simulink model "Half_3_Legs_with_RL_load"  (R2025b)
settings: Solver=VariableStepAuto  StartTime=0.0  StopTime=0.1  FixedStep=1e-6  MaxStep=1e-6  RelTol=1e-4
values from neighbouring files (symbols this model uses):
  bias_current = 5    [parameters_for_AMB_topology.m]
  half_SW_Ts = SW_Ts*0.5    (= 2.5e-05)    [parameters_for_AMB_topology.m]
  K_i = 2*pi*f_c*R_value/U_dc    (= 47.1238898038)    [parameters_for_AMB_topology.m]
  K_p = 2*pi*f_c*L_value/U_dc    (= 0.0235619449019)    [parameters_for_AMB_topology.m]
  R_value = 1    [parameters_for_AMB_topology.m]
  SW_Ts = 1/(SW_frequency)    (= 5e-05)    [parameters_for_AMB_topology.m]
libraries: fl_lib x48, simulink x35, nesl_utility x26, ee_lib x16, eeGeneralControl x10
(part 1 of 4)
settings Model: SimulationMode=accelerator  Creator=ubuntu  LastModifiedBy=ubuntu

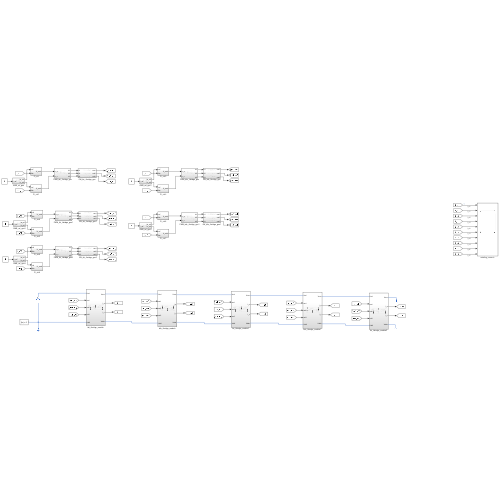
[thumbnail: Simulink's stored preview of the top-level diagram]
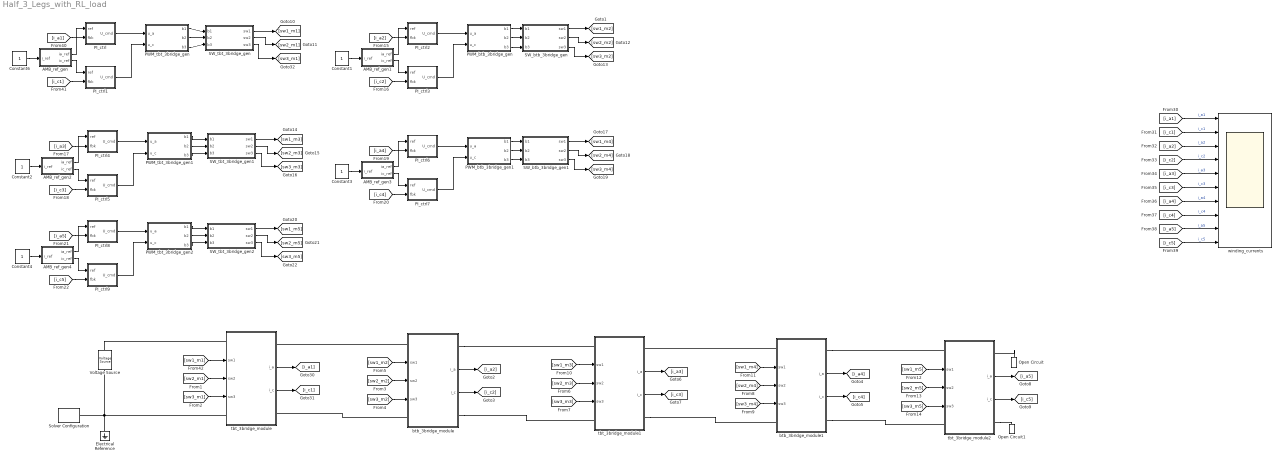
== system Half_3_Legs_with_RL_load ==
  AMB_ref_gen : Subsystem
  AMB_ref_gen1 : Subsystem
  AMB_ref_gen2 : Subsystem
  AMB_ref_gen3 : Subsystem
  AMB_ref_gen4 : Subsystem
  Constant{1..4,6} (5 alike) : Constant
  Electrical Reference : fl_lib/Electrical/Electrical Elements/Electrical Reference
  Open Circuit : fl_lib/Electrical/Electrical Elements/Open Circuit  v_specify=off  v_priority=None  v=0 V  v_nominal_specify=off  v_nominal_value=1  v_nominal_unit=V
  Open Circuit1 : fl_lib/Electrical/Electrical Elements/Open Circuit  v_specify=off  v_priority=None  v=0 V  v_nominal_specify=off  v_nominal_value=1  v_nominal_unit=V
  PI_ctrl : Subsystem
  PI_ctrl1 : Subsystem
  PI_ctrl2 : Subsystem
  PI_ctrl3 : Subsystem
  PI_ctrl4 : Subsystem
  PI_ctrl5 : Subsystem
  PI_ctrl6 : Subsystem
  PI_ctrl7 : Subsystem
  PI_ctrl8 : Subsystem
  PI_ctrl9 : Subsystem
  PWM_btb_3bridge_gen : Subsystem
  PWM_btb_3bridge_gen1 : Subsystem
  PWM_tbt_3bridge_gen : Subsystem
  PWM_tbt_3bridge_gen1 : Subsystem
  PWM_tbt_3bridge_gen2 : Subsystem
  SW_btb_3bridge_gen : Subsystem
  SW_btb_3bridge_gen1 : Subsystem
  SW_tbt_3bridge_gen : Subsystem
  SW_tbt_3bridge_gen1 : Subsystem
  SW_tbt_3bridge_gen2 : Subsystem
  Solver Configuration : nesl_utility/Solver Configuration  PhysicalDomain=network_engine_domain  SubClassName=solver  LeftPortType=input  RightPortType=generic  Tones=[]  Harmonics=[]  SimulateNoise=off  Profile=off  UseLocalSampling=off  EnableSwitchedLinearOptims=on  FrequencyDomain=off  UseCCode=off  RelTol=0.001  AbsTol=0.001  MinStep=1e-09  ToWorkspace=off  RevertToSquareIcSolve=off  NumHomotopyIterations=100  PhasorMode=off  PhasorModeNumHarmonics=1  ConsistencySolver=NEWTON_XTOL_AFTER_FTOL  IndexReductionMethod=DerivativeReplacement  DoDC=off  ResidualTolerance=1e-09  ConsistencyTolSource=GLOBAL  ConsistencyAbsTol=0.001  ConsistencyRelTol=0.001  ConsistencyTolFactor=0.001  UseLocalSolver=off  LocalSolverChoice=NE_TRAPEZOIDAL_ADVANCER  ResolveIndetEquations=on  FunctionEvalNumThread=1  LocalSolverSampleTime=1e-6  DoFixedCost=off  MaxNonlinIter=3  MaxModeIter=2  ComputeImpulses=off  ImpulseIterations=2  LinearAlgebra=auto  LinearAlgebraNumThread=0  EquationFormulation=NE_TIME_EF  DelaysMemoryBudget=1024  AutomaticFiltering=on  FilteringTimeConstant=0.001  PartitionStorageMethod=AS_NEEDED  PartitionMemoryBudget=1024  PartitionMethod=ROBUST  MultibodyUseLocalSolver=off  MultibodyLocalSolverChoice=ODE1  MultibodyLocalSolverSampleTime=0.001
  Voltage Source : ee_lib/Sources/Voltage Source  dc_voltage=U_dc V  ac_voltage=0 V  ac_shift=0 rad  ac_frequency=60 Hz  noise_mode=ee.enum.sources.noise.Disabled  PSD=0 V^2/Hz  sample_time=1e-3 s  repeatability=ee.enum.sources.repeatability.NotRepeatable  user_seed=0  auto_seed=3499211588  i_specify=off  i_priority=None  i=0 A  i_nominal_specify=off  i_nominal_value=1  i_nominal_unit=A  v_specify=off  v_priority=None  v=0 V  v_nominal_specify=off  v_nominal_value=1  v_nominal_unit=V
  btb_3bridge_module : Subsystem
      settings: PortSchema="{\"entries\":[{\"content\":{\"sides\":[{\"content\":{\"connectorIds\":[\"LConn1\",\"In1\",\"In2\",\"In3\",\"LConn2\"]},\"type\":\"ConnectorPlacement.EquallySpacedRectSide\",\"uuid\":\"10840d64-2819-4406-b8bd-231f9b995eba\"},{\"content\":{\"connectorIds\":[\"RConn1\",\"Out1\",\"Out2\",\"RConn2\"],\"side\":\"RIGHT\"},\"type\":\"ConnectorPlacement.EquallySpacedRectSide\",\"uuid\":\"cbdb59db-7701-4ec8-b1d6-0cae4f1e7bab\"},{\"content\":{\"side\":\"TOP\"},\"type\":\"ConnectorPlacement.EquallySpacedRectSide\",\"uuid\":\"7d2d29df-036d-4b8e-bd54-59e76fc95f5a\"}]},\"type\":\"ConnectorPlacement.EquallySpacedConnector\",\"uuid\":\"03b861fb-a6f3-4cde-b4d6-1419ababfbe2\"}],\"packageUris\":[\"http://schema.mathworks.com/mf0/Connector/R2020b\"],\"version\":\"1.0\"}"
  btb_3bridge_module1 : Subsystem
      settings: PortSchema="{\"entries\":[{\"content\":{\"sides\":[{\"content\":{\"connectorIds\":[\"LConn1\",\"In1\",\"In2\",\"In3\",\"LConn2\"]},\"type\":\"ConnectorPlacement.EquallySpacedRectSide\",\"uuid\":\"10840d64-2819-4406-b8bd-231f9b995eba\"},{\"content\":{\"connectorIds\":[\"RConn1\",\"Out1\",\"Out2\",\"RConn2\"],\"side\":\"RIGHT\"},\"type\":\"ConnectorPlacement.EquallySpacedRectSide\",\"uuid\":\"cbdb59db-7701-4ec8-b1d6-0cae4f1e7bab\"},{\"content\":{\"side\":\"TOP\"},\"type\":\"ConnectorPlacement.EquallySpacedRectSide\",\"uuid\":\"7d2d29df-036d-4b8e-bd54-59e76fc95f5a\"}]},\"type\":\"ConnectorPlacement.EquallySpacedConnector\",\"uuid\":\"03b861fb-a6f3-4cde-b4d6-1419ababfbe2\"}],\"packageUris\":[\"http://schema.mathworks.com/mf0/Connector/R2020b\"],\"version\":\"1.0\"}"
  tbt_3bridge_module : Subsystem
      settings: PortSchema="{\"entries\":[{\"content\":{\"sides\":[{\"content\":{\"connectorIds\":[\"LConn1\",\"In1\",\"In2\",\"In3\",\"LConn2\"]},\"type\":\"ConnectorPlacement.EquallySpacedRectSide\",\"uuid\":\"10840d64-2819-4406-b8bd-231f9b995eba\"},{\"content\":{\"connectorIds\":[\"RConn1\",\"Out1\",\"Out2\",\"RConn2\"],\"side\":\"RIGHT\"},\"type\":\"ConnectorPlacement.EquallySpacedRectSide\",\"uuid\":\"cbdb59db-7701-4ec8-b1d6-0cae4f1e7bab\"},{\"content\":{\"side\":\"TOP\"},\"type\":\"ConnectorPlacement.EquallySpacedRectSide\",\"uuid\":\"7d2d29df-036d-4b8e-bd54-59e76fc95f5a\"}]},\"type\":\"ConnectorPlacement.EquallySpacedConnector\",\"uuid\":\"03b861fb-a6f3-4cde-b4d6-1419ababfbe2\"}],\"packageUris\":[\"http://schema.mathworks.com/mf0/Connector/R2020b\"],\"version\":\"1.0\"}"
  tbt_3bridge_module1 : Subsystem
      settings: PortSchema="{\"entries\":[{\"content\":{\"sides\":[{\"content\":{\"connectorIds\":[\"LConn1\",\"In1\",\"In2\",\"In3\",\"LConn2\"]},\"type\":\"ConnectorPlacement.EquallySpacedRectSide\",\"uuid\":\"10840d64-2819-4406-b8bd-231f9b995eba\"},{\"content\":{\"connectorIds\":[\"RConn1\",\"Out1\",\"Out2\",\"RConn2\"],\"side\":\"RIGHT\"},\"type\":\"ConnectorPlacement.EquallySpacedRectSide\",\"uuid\":\"cbdb59db-7701-4ec8-b1d6-0cae4f1e7bab\"},{\"content\":{\"side\":\"TOP\"},\"type\":\"ConnectorPlacement.EquallySpacedRectSide\",\"uuid\":\"7d2d29df-036d-4b8e-bd54-59e76fc95f5a\"}]},\"type\":\"ConnectorPlacement.EquallySpacedConnector\",\"uuid\":\"03b861fb-a6f3-4cde-b4d6-1419ababfbe2\"}],\"packageUris\":[\"http://schema.mathworks.com/mf0/Connector/R2020b\"],\"version\":\"1.0\"}"
  tbt_3bridge_module2 : Subsystem
      settings: PortSchema="{\"entries\":[{\"content\":{\"sides\":[{\"content\":{\"connectorIds\":[\"LConn1\",\"In1\",\"In2\",\"In3\",\"LConn2\"]},\"type\":\"ConnectorPlacement.EquallySpacedRectSide\",\"uuid\":\"10840d64-2819-4406-b8bd-231f9b995eba\"},{\"content\":{\"connectorIds\":[\"RConn1\",\"Out1\",\"Out2\",\"RConn2\"],\"side\":\"RIGHT\"},\"type\":\"ConnectorPlacement.EquallySpacedRectSide\",\"uuid\":\"cbdb59db-7701-4ec8-b1d6-0cae4f1e7bab\"},{\"content\":{\"side\":\"TOP\"},\"type\":\"ConnectorPlacement.EquallySpacedRectSide\",\"uuid\":\"7d2d29df-036d-4b8e-bd54-59e76fc95f5a\"}]},\"type\":\"ConnectorPlacement.EquallySpacedConnector\",\"uuid\":\"03b861fb-a6f3-4cde-b4d6-1419ababfbe2\"}],\"packageUris\":[\"http://schema.mathworks.com/mf0/Connector/R2020b\"],\"version\":\"1.0\"}"
  winding_currents : Scope  NumInputPorts=10
      settings: ActiveDisplayYMinimum=-0.73222271304047026  ActiveDisplayYMaximum=6.5900064127702036
  wires:
  [i_a1] -> winding_currents/1  "i_a1"
  [i_c1] -> winding_currents/2  "i_c1"
  [i_a2] -> winding_currents/3  "i_a2"
  [i_c2] -> winding_currents/4  "i_c2"
  [i_a3] -> winding_currents/5  "i_a3"
  [i_c3] -> winding_currents/6  "i_c3"
  [i_a4] -> winding_currents/7  "i_a4"
  [i_c4] -> winding_currents/8  "i_c4"
  [i_a5] -> winding_currents/9  "i_a5"
  [i_c5] -> winding_currents/10  "i_c5"
  AMB_ref_gen/1(ia_ref) -> PI_ctrl/1(ref)
  AMB_ref_gen/2(ic_ref) -> PI_ctrl1/1(ref)
  Constant6/1 -> AMB_ref_gen/1(i_ref)
  [i_a1] -> PI_ctrl/2(fbk)
  [i_c1] -> PI_ctrl1/2(fbk)
  PI_ctrl/1(U_cmd) -> PWM_tbt_3bridge_gen/1(u_a)
  PI_ctrl1/1(U_cmd) -> PWM_tbt_3bridge_gen/2(u_c)
  PWM_tbt_3bridge_gen/1(b1) -> SW_tbt_3bridge_gen/1(b1)
  PWM_tbt_3bridge_gen/2(b2) -> SW_tbt_3bridge_gen/2(b2)
  PWM_tbt_3bridge_gen/3(b3) -> SW_tbt_3bridge_gen/3(b3)
  tbt_3bridge_module/1(i_a) -> [i_a1]
  tbt_3bridge_module/2(i_c) -> [i_c1]
  [sw1_m1] -> tbt_3bridge_module/1(sw1)
  [sw2_m1] -> tbt_3bridge_module/2(sw2)
  [sw3_m1] -> tbt_3bridge_module/3(sw3)
  [sw1_m2] -> btb_3bridge_module/1(sw1)
  [sw3_m2] -> btb_3bridge_module/3(sw3)
  [sw2_m2] -> btb_3bridge_module/2(sw2)
  btb_3bridge_module/1(i_a) -> [i_a2]
  btb_3bridge_module/2(i_c) -> [i_c2]
  [sw2_m4] -> btb_3bridge_module1/2(sw2)
  btb_3bridge_module1/1(i_a) -> [i_a4]
  [sw2_m3] -> tbt_3bridge_module1/2(sw2)
  [sw1_m4] -> btb_3bridge_module1/1(sw1)
  [sw1_m3] -> tbt_3bridge_module1/1(sw1)
  [sw3_m3] -> tbt_3bridge_module1/3(sw3)
  btb_3bridge_module1/2(i_c) -> [i_c4]
  [sw3_m4] -> btb_3bridge_module1/3(sw3)
  tbt_3bridge_module1/2(i_c) -> [i_c3]
  tbt_3bridge_module1/1(i_a) -> [i_a3]
  tbt_3bridge_module2/2(i_c) -> [i_c5]
  [sw3_m5] -> tbt_3bridge_module2/3(sw3)
  [sw2_m5] -> tbt_3bridge_module2/2(sw2)
  [sw1_m5] -> tbt_3bridge_module2/1(sw1)
  tbt_3bridge_module2/1(i_a) -> [i_a5]
  SW_tbt_3bridge_gen/1(sw1) -> [sw1_m1]
  SW_tbt_3bridge_gen/2(sw2) -> [sw2_m1]
  SW_tbt_3bridge_gen/3(sw3) -> [sw3_m1]
  [i_c2] -> PI_ctrl3/2(fbk)
  SW_btb_3bridge_gen/2(sw2) -> [sw2_m2]
  PWM_btb_3bridge_gen/2(b2) -> SW_btb_3bridge_gen/2(b2)
  PI_ctrl2/1(U_cmd) -> PWM_btb_3bridge_gen/1(u_a)
  AMB_ref_gen1/2(ic_ref) -> PI_ctrl3/1(ref)
  PWM_btb_3bridge_gen/1(b1) -> SW_btb_3bridge_gen/1(b1)
  AMB_ref_gen1/1(ia_ref) -> PI_ctrl2/1(ref)
  SW_btb_3bridge_gen/1(sw1) -> [sw1_m2]
  SW_btb_3bridge_gen/3(sw3) -> [sw3_m2]
  PI_ctrl3/1(U_cmd) -> PWM_btb_3bridge_gen/2(u_c)
  PWM_btb_3bridge_gen/3(b3) -> SW_btb_3bridge_gen/3(b3)
  [i_a2] -> PI_ctrl2/2(fbk)
  Constant1/1 -> AMB_ref_gen1/1(i_ref)
  [i_c3] -> PI_ctrl5/2(fbk)
  SW_tbt_3bridge_gen1/2(sw2) -> [sw2_m3]
  PWM_tbt_3bridge_gen1/2(b2) -> SW_tbt_3bridge_gen1/2(b2)
  PI_ctrl4/1(U_cmd) -> PWM_tbt_3bridge_gen1/1(u_a)
  AMB_ref_gen2/2(ic_ref) -> PI_ctrl5/1(ref)
  PWM_tbt_3bridge_gen1/1(b1) -> SW_tbt_3bridge_gen1/1(b1)
  AMB_ref_gen2/1(ia_ref) -> PI_ctrl4/1(ref)
  SW_tbt_3bridge_gen1/1(sw1) -> [sw1_m3]
  SW_tbt_3bridge_gen1/3(sw3) -> [sw3_m3]
  PI_ctrl5/1(U_cmd) -> PWM_tbt_3bridge_gen1/2(u_c)
  PWM_tbt_3bridge_gen1/3(b3) -> SW_tbt_3bridge_gen1/3(b3)
  [i_a3] -> PI_ctrl4/2(fbk)
  Constant2/1 -> AMB_ref_gen2/1(i_ref)
  AMB_ref_gen3/2(ic_ref) -> PI_ctrl7/1(ref)
  PWM_btb_3bridge_gen1/3(b3) -> SW_btb_3bridge_gen1/3(b3)
  SW_btb_3bridge_gen1/1(sw1) -> [sw1_m4]
  PWM_btb_3bridge_gen1/1(b1) -> SW_btb_3bridge_gen1/1(b1)
  SW_btb_3bridge_gen1/2(sw2) -> [sw2_m4]
  [i_c4] -> PI_ctrl7/2(fbk)
  AMB_ref_gen3/1(ia_ref) -> PI_ctrl6/1(ref)
  [i_a4] -> PI_ctrl6/2(fbk)
  SW_btb_3bridge_gen1/3(sw3) -> [sw3_m4]
  PWM_btb_3bridge_gen1/2(b2) -> SW_btb_3bridge_gen1/2(b2)
  PI_ctrl6/1(U_cmd) -> PWM_btb_3bridge_gen1/1(u_a)
  Constant3/1 -> AMB_ref_gen3/1(i_ref)
  PI_ctrl7/1(U_cmd) -> PWM_btb_3bridge_gen1/2(u_c)
  PWM_tbt_3bridge_gen2/2(b2) -> SW_tbt_3bridge_gen2/2(b2)
  PI_ctrl8/1(U_cmd) -> PWM_tbt_3bridge_gen2/1(u_a)
  SW_tbt_3bridge_gen2/1(sw1) -> [sw1_m5]
  [i_c5] -> PI_ctrl9/2(fbk)
  AMB_ref_gen4/2(ic_ref) -> PI_ctrl9/1(ref)
  PWM_tbt_3bridge_gen2/1(b1) -> SW_tbt_3bridge_gen2/1(b1)
  PWM_tbt_3bridge_gen2/3(b3) -> SW_tbt_3bridge_gen2/3(b3)
  AMB_ref_gen4/1(ia_ref) -> PI_ctrl8/1(ref)
  Constant4/1 -> AMB_ref_gen4/1(i_ref)
  PI_ctrl9/1(U_cmd) -> PWM_tbt_3bridge_gen2/2(u_c)
  SW_tbt_3bridge_gen2/3(sw3) -> [sw3_m5]
  [i_a5] -> PI_ctrl8/2(fbk)
  SW_tbt_3bridge_gen2/2(sw2) -> [sw2_m5]
  connections:
  Electrical Reference/LConn1 -- Voltage Source/RConn1 -- tbt_3bridge_module/LConn2 -- Solver Configuration/RConn1
  tbt_3bridge_module/LConn1 -- Voltage Source/LConn1
  btb_3bridge_module/LConn1 -- tbt_3bridge_module/RConn1
  btb_3bridge_module/LConn2 -- tbt_3bridge_module/RConn2
  btb_3bridge_module/RConn1 -- tbt_3bridge_module1/LConn1
  btb_3bridge_module/RConn2 -- tbt_3bridge_module1/LConn2
  btb_3bridge_module1/LConn1 -- tbt_3bridge_module1/RConn1
  tbt_3bridge_module1/RConn2 -- btb_3bridge_module1/LConn2
  btb_3bridge_module1/RConn1 -- tbt_3bridge_module2/LConn1
  btb_3bridge_module1/RConn2 -- tbt_3bridge_module2/LConn2
  Open Circuit/LConn1 -- tbt_3bridge_module2/RConn1
  tbt_3bridge_module2/RConn2 -- Open Circuit1/LConn1

== system Half_3_Legs_with_RL_load/AMB_ref_gen ==
  i_ref : Inport
  Add : Sum
  Add1 : Sum  Inputs=-+
  Constant : Constant  Value=bias_current
  Gain : Gain  Gain=0.5
  ia_ref : Outport
  ic_ref : Outport  Port=2
  wires:
  i_ref/1 -> Gain/1
  Gain/1 -> Add1/1, Add/2
  Add/1 -> ia_ref/1
  Constant/1 -> Add1/2, Add/1
  Add1/1 -> ic_ref/1

== system Half_3_Legs_with_RL_load/AMB_ref_gen1 ==
  i_ref : Inport
  Add : Sum
  Add1 : Sum  Inputs=-+
  Constant : Constant  Value=bias_current
  Gain : Gain  Gain=0.5
  ia_ref : Outport
  ic_ref : Outport  Port=2
  wires:
  i_ref/1 -> Gain/1
  Gain/1 -> Add1/1, Add/2
  Add/1 -> ia_ref/1
  Constant/1 -> Add1/2, Add/1
  Add1/1 -> ic_ref/1

== system Half_3_Legs_with_RL_load/AMB_ref_gen2 ==
  i_ref : Inport
  Add : Sum
  Add1 : Sum  Inputs=-+
  Constant : Constant  Value=bias_current
  Gain : Gain  Gain=0.5
  ia_ref : Outport
  ic_ref : Outport  Port=2
  wires:
  i_ref/1 -> Gain/1
  Gain/1 -> Add1/1, Add/2
  Add/1 -> ia_ref/1
  Constant/1 -> Add1/2, Add/1
  Add1/1 -> ic_ref/1

== system Half_3_Legs_with_RL_load/AMB_ref_gen3 ==
  i_ref : Inport
  Add : Sum
  Add1 : Sum  Inputs=-+
  Constant : Constant  Value=bias_current
  Gain : Gain  Gain=0.5
  ia_ref : Outport
  ic_ref : Outport  Port=2
  wires:
  i_ref/1 -> Gain/1
  Gain/1 -> Add1/1, Add/2
  Add/1 -> ia_ref/1
  Constant/1 -> Add1/2, Add/1
  Add1/1 -> ic_ref/1

== system Half_3_Legs_with_RL_load/AMB_ref_gen4 ==
  i_ref : Inport
  Add : Sum
  Add1 : Sum  Inputs=-+
  Constant : Constant  Value=bias_current
  Gain : Gain  Gain=0.5
  ia_ref : Outport
  ic_ref : Outport  Port=2
  wires:
  i_ref/1 -> Gain/1
  Gain/1 -> Add1/1, Add/2
  Add/1 -> ia_ref/1
  Constant/1 -> Add1/2, Add/1
  Add1/1 -> ic_ref/1

== system Half_3_Legs_with_RL_load/PI_ctrl ==
  ref : Inport
  fbk : Inport  Port=2
  Add2 : Sum  Inputs=+-
  Add3 : Sum
  Gain4 : Gain  Gain=K_p
  Ictrl_anti_windup : Subsystem
  Memory : Memory
  Rate Transition : RateTransition  OutPortSampleTime=SW_Ts
  Saturation : Saturate  UpperLimit=1  LowerLimit=-1
  Second-Order Filter : eeGeneralControl/Second-Order Filter  FilterType=Low-pass  fn=6000  Zeta=0.707  Ts=0  A0=0  Ph0=0  f0=0  b0=0
      settings: LibrarySourceBlock=ee_sl_lib/General Control/Second-Order Filter
  U_cmd : Outport
  wires:
  Gain4/1 -> Add3/1
  Memory/1 -> Second-Order Filter/1
  Second-Order Filter/1 -> Add2/2
  Saturation/1 -> U_cmd/1
  Add2/1 -> Ictrl_anti_windup/1(err), Gain4/1
  Add3/1 -> Saturation/1
  ref/1 -> Add2/1
  fbk/1 -> Rate Transition/1
  Rate Transition/1 -> Memory/1
  Ictrl_anti_windup/1(Int_out) -> Add3/2

== system Half_3_Legs_with_RL_load/PI_ctrl1 ==
  ref : Inport
  fbk : Inport  Port=2
  Add2 : Sum  Inputs=+-
  Add3 : Sum
  Gain4 : Gain  Gain=K_p
  Ictrl_anti_windup : Subsystem
  Memory : Memory
  Rate Transition : RateTransition  OutPortSampleTime=SW_Ts
  Saturation : Saturate  UpperLimit=1  LowerLimit=-1
  Second-Order Filter : eeGeneralControl/Second-Order Filter  FilterType=Low-pass  fn=6000  Zeta=0.707  Ts=0  A0=0  Ph0=0  f0=0  b0=0
      settings: LibrarySourceBlock=ee_sl_lib/General Control/Second-Order Filter
  U_cmd : Outport
  wires:
  Gain4/1 -> Add3/1
  Memory/1 -> Second-Order Filter/1
  Second-Order Filter/1 -> Add2/2
  Saturation/1 -> U_cmd/1
  Add2/1 -> Ictrl_anti_windup/1(err), Gain4/1
  Add3/1 -> Saturation/1
  ref/1 -> Add2/1
  fbk/1 -> Rate Transition/1
  Rate Transition/1 -> Memory/1
  Ictrl_anti_windup/1(Int_out) -> Add3/2

== system Half_3_Legs_with_RL_load/PI_ctrl2 ==
  ref : Inport
  fbk : Inport  Port=2
  Add2 : Sum  Inputs=+-
  Add3 : Sum
  Gain4 : Gain  Gain=K_p
  Ictrl_anti_windup : Subsystem
  Memory : Memory
  Rate Transition : RateTransition  OutPortSampleTime=SW_Ts
  Saturation : Saturate  UpperLimit=1  LowerLimit=-1
  Second-Order Filter : eeGeneralControl/Second-Order Filter  FilterType=Low-pass  fn=6000  Zeta=0.707  Ts=0  A0=0  Ph0=0  f0=0  b0=0
      settings: LibrarySourceBlock=ee_sl_lib/General Control/Second-Order Filter
  U_cmd : Outport
  wires:
  Gain4/1 -> Add3/1
  Memory/1 -> Second-Order Filter/1
  Second-Order Filter/1 -> Add2/2
  Saturation/1 -> U_cmd/1
  Add2/1 -> Ictrl_anti_windup/1(err), Gain4/1
  Add3/1 -> Saturation/1
  ref/1 -> Add2/1
  fbk/1 -> Rate Transition/1
  Rate Transition/1 -> Memory/1
  Ictrl_anti_windup/1(Int_out) -> Add3/2

== system Half_3_Legs_with_RL_load/PI_ctrl3 ==
  ref : Inport
  fbk : Inport  Port=2
  Add2 : Sum  Inputs=+-
  Add3 : Sum
  Gain4 : Gain  Gain=K_p
  Ictrl_anti_windup : Subsystem
  Memory : Memory
  Rate Transition : RateTransition  OutPortSampleTime=SW_Ts
  Saturation : Saturate  UpperLimit=1  LowerLimit=-1
  Second-Order Filter : eeGeneralControl/Second-Order Filter  FilterType=Low-pass  fn=6000  Zeta=0.707  Ts=0  A0=0  Ph0=0  f0=0  b0=0
      settings: LibrarySourceBlock=ee_sl_lib/General Control/Second-Order Filter
  U_cmd : Outport
  wires:
  Gain4/1 -> Add3/1
  Memory/1 -> Second-Order Filter/1
  Second-Order Filter/1 -> Add2/2
  Saturation/1 -> U_cmd/1
  Add2/1 -> Ictrl_anti_windup/1(err), Gain4/1
  Add3/1 -> Saturation/1
  ref/1 -> Add2/1
  fbk/1 -> Rate Transition/1
  Rate Transition/1 -> Memory/1
  Ictrl_anti_windup/1(Int_out) -> Add3/2

== system Half_3_Legs_with_RL_load/PI_ctrl4 ==
  ref : Inport
  fbk : Inport  Port=2
  Add2 : Sum  Inputs=+-
  Add3 : Sum
  Gain4 : Gain  Gain=K_p
  Ictrl_anti_windup : Subsystem
  Memory : Memory
  Rate Transition : RateTransition  OutPortSampleTime=SW_Ts
  Saturation : Saturate  UpperLimit=1  LowerLimit=-1
  Second-Order Filter : eeGeneralControl/Second-Order Filter  FilterType=Low-pass  fn=6000  Zeta=0.707  Ts=0  A0=0  Ph0=0  f0=0  b0=0
      settings: LibrarySourceBlock=ee_sl_lib/General Control/Second-Order Filter
  U_cmd : Outport
  wires:
  Gain4/1 -> Add3/1
  Memory/1 -> Second-Order Filter/1
  Second-Order Filter/1 -> Add2/2
  Saturation/1 -> U_cmd/1
  Add2/1 -> Ictrl_anti_windup/1(err), Gain4/1
  Add3/1 -> Saturation/1
  ref/1 -> Add2/1
  fbk/1 -> Rate Transition/1
  Rate Transition/1 -> Memory/1
  Ictrl_anti_windup/1(Int_out) -> Add3/2

== system Half_3_Legs_with_RL_load/PI_ctrl5 ==
  ref : Inport
  fbk : Inport  Port=2
  Add2 : Sum  Inputs=+-
  Add3 : Sum
  Gain4 : Gain  Gain=K_p
  Ictrl_anti_windup : Subsystem
  Memory : Memory
  Rate Transition : RateTransition  OutPortSampleTime=SW_Ts
  Saturation : Saturate  UpperLimit=1  LowerLimit=-1
  Second-Order Filter : eeGeneralControl/Second-Order Filter  FilterType=Low-pass  fn=6000  Zeta=0.707  Ts=0  A0=0  Ph0=0  f0=0  b0=0
      settings: LibrarySourceBlock=ee_sl_lib/General Control/Second-Order Filter
  U_cmd : Outport
  wires:
  Gain4/1 -> Add3/1
  Memory/1 -> Second-Order Filter/1
  Second-Order Filter/1 -> Add2/2
  Saturation/1 -> U_cmd/1
  Add2/1 -> Ictrl_anti_windup/1(err), Gain4/1
  Add3/1 -> Saturation/1
  ref/1 -> Add2/1
  fbk/1 -> Rate Transition/1
  Rate Transition/1 -> Memory/1
  Ictrl_anti_windup/1(Int_out) -> Add3/2

== system Half_3_Legs_with_RL_load/PI_ctrl6 ==
  ref : Inport
  fbk : Inport  Port=2
  Add2 : Sum  Inputs=+-
  Add3 : Sum
  Gain4 : Gain  Gain=K_p
  Ictrl_anti_windup : Subsystem
  Memory : Memory
  Rate Transition : RateTransition  OutPortSampleTime=SW_Ts
  Saturation : Saturate  UpperLimit=1  LowerLimit=-1
  Second-Order Filter : eeGeneralControl/Second-Order Filter  FilterType=Low-pass  fn=6000  Zeta=0.707  Ts=0  A0=0  Ph0=0  f0=0  b0=0
      settings: LibrarySourceBlock=ee_sl_lib/General Control/Second-Order Filter
  U_cmd : Outport
  wires:
  Gain4/1 -> Add3/1
  Memory/1 -> Second-Order Filter/1
  Second-Order Filter/1 -> Add2/2
  Saturation/1 -> U_cmd/1
  Add2/1 -> Ictrl_anti_windup/1(err), Gain4/1
  Add3/1 -> Saturation/1
  ref/1 -> Add2/1
  fbk/1 -> Rate Transition/1
  Rate Transition/1 -> Memory/1
  Ictrl_anti_windup/1(Int_out) -> Add3/2

== system Half_3_Legs_with_RL_load/PI_ctrl7 ==
  ref : Inport
  fbk : Inport  Port=2
  Add2 : Sum  Inputs=+-
  Add3 : Sum
  Gain4 : Gain  Gain=K_p
  Ictrl_anti_windup : Subsystem
  Memory : Memory
  Rate Transition : RateTransition  OutPortSampleTime=SW_Ts
  Saturation : Saturate  UpperLimit=1  LowerLimit=-1
  Second-Order Filter : eeGeneralControl/Second-Order Filter  FilterType=Low-pass  fn=6000  Zeta=0.707  Ts=0  A0=0  Ph0=0  f0=0  b0=0
      settings: LibrarySourceBlock=ee_sl_lib/General Control/Second-Order Filter
  U_cmd : Outport
  wires:
  Gain4/1 -> Add3/1
  Memory/1 -> Second-Order Filter/1
  Second-Order Filter/1 -> Add2/2
  Saturation/1 -> U_cmd/1
  Add2/1 -> Ictrl_anti_windup/1(err), Gain4/1
  Add3/1 -> Saturation/1
  ref/1 -> Add2/1
  fbk/1 -> Rate Transition/1
  Rate Transition/1 -> Memory/1
  Ictrl_anti_windup/1(Int_out) -> Add3/2

== system Half_3_Legs_with_RL_load/PI_ctrl8 ==
  ref : Inport
  fbk : Inport  Port=2
  Add2 : Sum  Inputs=+-
  Add3 : Sum
  Gain4 : Gain  Gain=K_p
  Ictrl_anti_windup : Subsystem
  Memory : Memory
  Rate Transition : RateTransition  OutPortSampleTime=SW_Ts
  Saturation : Saturate  UpperLimit=1  LowerLimit=-1
  Second-Order Filter : eeGeneralControl/Second-Order Filter  FilterType=Low-pass  fn=6000  Zeta=0.707  Ts=0  A0=0  Ph0=0  f0=0  b0=0
      settings: LibrarySourceBlock=ee_sl_lib/General Control/Second-Order Filter
  U_cmd : Outport
  wires:
  Gain4/1 -> Add3/1
  Memory/1 -> Second-Order Filter/1
  Second-Order Filter/1 -> Add2/2
  Saturation/1 -> U_cmd/1
  Add2/1 -> Ictrl_anti_windup/1(err), Gain4/1
  Add3/1 -> Saturation/1
  ref/1 -> Add2/1
  fbk/1 -> Rate Transition/1
  Rate Transition/1 -> Memory/1
  Ictrl_anti_windup/1(Int_out) -> Add3/2

== system Half_3_Legs_with_RL_load/PI_ctrl9 ==
  ref : Inport
  fbk : Inport  Port=2
  Add2 : Sum  Inputs=+-
  Add3 : Sum
  Gain4 : Gain  Gain=K_p
  Ictrl_anti_windup : Subsystem
  Memory : Memory
  Rate Transition : RateTransition  OutPortSampleTime=SW_Ts
  Saturation : Saturate  UpperLimit=1  LowerLimit=-1
  Second-Order Filter : eeGeneralControl/Second-Order Filter  FilterType=Low-pass  fn=6000  Zeta=0.707  Ts=0  A0=0  Ph0=0  f0=0  b0=0
      settings: LibrarySourceBlock=ee_sl_lib/General Control/Second-Order Filter
  U_cmd : Outport
  wires:
  Gain4/1 -> Add3/1
  Memory/1 -> Second-Order Filter/1
  Second-Order Filter/1 -> Add2/2
  Saturation/1 -> U_cmd/1
  Add2/1 -> Ictrl_anti_windup/1(err), Gain4/1
  Add3/1 -> Saturation/1
  ref/1 -> Add2/1
  fbk/1 -> Rate Transition/1
  Rate Transition/1 -> Memory/1
  Ictrl_anti_windup/1(Int_out) -> Add3/2

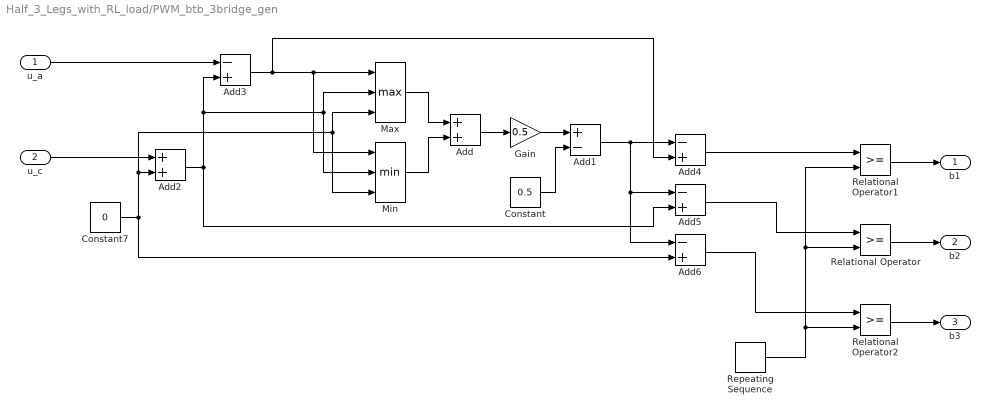
== system Half_3_Legs_with_RL_load/PWM_btb_3bridge_gen ==
  u_a : Inport
  u_c : Inport  Port=2
  Add : Sum
  Add1 : Sum  Inputs=+-
  Add2 : Sum
  Add{3..6} (4 alike) : Sum  Inputs=-+
  Constant : Constant  Value=0.5
  Constant7 : Constant  Value=0
  Gain : Gain  Gain=0.5
  Max : MinMax  Function=max  Inputs=3
  Min : MinMax  Inputs=3
  Relational Operator : RelationalOperator  OutDataTypeStr=boolean  RndMeth=Simplest  InputSameDT=off
  Relational Operator1 : RelationalOperator  OutDataTypeStr=boolean  RndMeth=Simplest  InputSameDT=off
  Relational Operator2 : RelationalOperator  OutDataTypeStr=boolean  RndMeth=Simplest  InputSameDT=off
  Repeating Sequence : simulink/Sources/Repeating Sequence  rep_seq_t=[0 half_SW_Ts SW_Ts]  rep_seq_y=[0 1 0]
  b1 : Outport
  b2 : Outport  Port=2
  b3 : Outport  Port=3
  wires:
  Add4/1 -> Relational Operator1/1
  Max/1 -> Add/1
  Gain/1 -> Add1/1
  u_c/1 -> Add2/1
  Relational Operator2/1 -> b3/1
  Min/1 -> Add/2
  Relational Operator1/1 -> b1/1
  Constant/1 -> Add1/2
  Add3/1 -> Add4/2, Min/1, Max/1
  Relational Operator/1 -> b2/1
  Add2/1 -> Add5/2, Min/2, Max/2, Add3/2
  u_a/1 -> Add3/1
  Add1/1 -> Add6/1, Add5/1, Add4/1
  Add6/1 -> Relational Operator2/1
  Repeating Sequence/1 -> Relational Operator2/2, Relational Operator1/2, Relational Operator/2
  Constant7/1 -> Add6/2, Min/3, Max/3, Add2/2
  Add/1 -> Gain/1
  Add5/1 -> Relational Operator/1

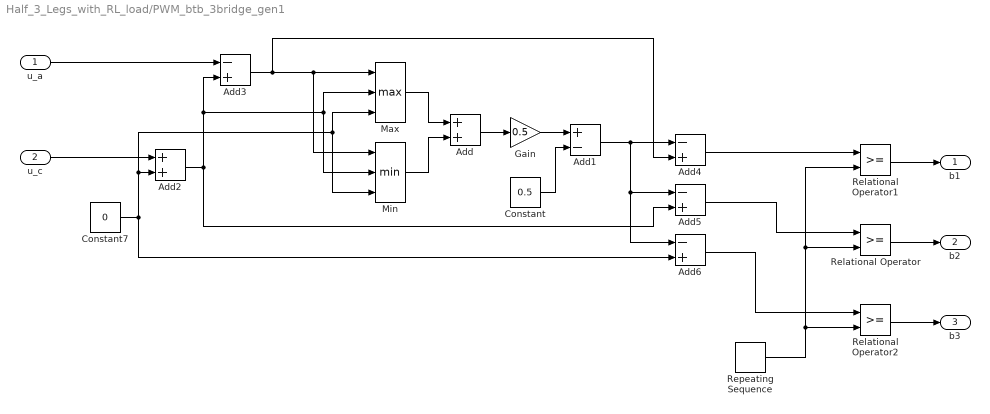
== system Half_3_Legs_with_RL_load/PWM_btb_3bridge_gen1 ==
  u_a : Inport
  u_c : Inport  Port=2
  Add : Sum
  Add1 : Sum  Inputs=+-
  Add2 : Sum
  Add{3..6} (4 alike) : Sum  Inputs=-+
  Constant : Constant  Value=0.5
  Constant7 : Constant  Value=0
  Gain : Gain  Gain=0.5
  Max : MinMax  Function=max  Inputs=3
  Min : MinMax  Inputs=3
  Relational Operator : RelationalOperator  OutDataTypeStr=boolean  RndMeth=Simplest  InputSameDT=off
  Relational Operator1 : RelationalOperator  OutDataTypeStr=boolean  RndMeth=Simplest  InputSameDT=off
  Relational Operator2 : RelationalOperator  OutDataTypeStr=boolean  RndMeth=Simplest  InputSameDT=off
  Repeating Sequence : simulink/Sources/Repeating Sequence  rep_seq_t=[0 half_SW_Ts SW_Ts]  rep_seq_y=[0 1 0]
  b1 : Outport
  b2 : Outport  Port=2
  b3 : Outport  Port=3
  wires:
  Add4/1 -> Relational Operator1/1
  Max/1 -> Add/1
  Gain/1 -> Add1/1
  u_c/1 -> Add2/1
  Relational Operator2/1 -> b3/1
  Min/1 -> Add/2
  Relational Operator1/1 -> b1/1
  Constant/1 -> Add1/2
  Add3/1 -> Add4/2, Min/1, Max/1
  Relational Operator/1 -> b2/1
  Add2/1 -> Add5/2, Min/2, Max/2, Add3/2
  u_a/1 -> Add3/1
  Add1/1 -> Add6/1, Add5/1, Add4/1
  Add6/1 -> Relational Operator2/1
  Repeating Sequence/1 -> Relational Operator2/2, Relational Operator1/2, Relational Operator/2
  Constant7/1 -> Add6/2, Min/3, Max/3, Add2/2
  Add/1 -> Gain/1
  Add5/1 -> Relational Operator/1

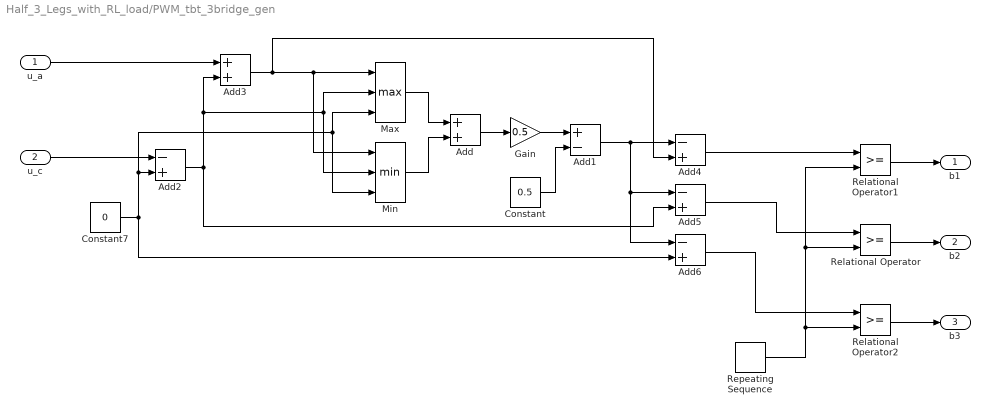
== system Half_3_Legs_with_RL_load/PWM_tbt_3bridge_gen ==
  u_a : Inport
  u_c : Inport  Port=2
  Add : Sum
  Add1 : Sum  Inputs=+-
  Add{2,4..6} (4 alike) : Sum  Inputs=-+
  Add3 : Sum
  Constant : Constant  Value=0.5
  Constant7 : Constant  Value=0
  Gain : Gain  Gain=0.5
  Max : MinMax  Function=max  Inputs=3
  Min : MinMax  Inputs=3
  Relational Operator : RelationalOperator  OutDataTypeStr=boolean  RndMeth=Simplest  InputSameDT=off
  Relational Operator1 : RelationalOperator  OutDataTypeStr=boolean  RndMeth=Simplest  InputSameDT=off
  Relational Operator2 : RelationalOperator  OutDataTypeStr=boolean  RndMeth=Simplest  InputSameDT=off
  Repeating Sequence : simulink/Sources/Repeating Sequence  rep_seq_t=[0 half_SW_Ts SW_Ts]  rep_seq_y=[0 1 0]
  b1 : Outport
  b2 : Outport  Port=2
  b3 : Outport  Port=3
  wires:
  Add4/1 -> Relational Operator1/1
  Max/1 -> Add/1
  Gain/1 -> Add1/1
  u_c/1 -> Add2/1
  Relational Operator2/1 -> b3/1
  Min/1 -> Add/2
  Relational Operator1/1 -> b1/1
  Constant/1 -> Add1/2
  Add3/1 -> Add4/2, Min/1, Max/1
  Relational Operator/1 -> b2/1
  Add2/1 -> Add5/2, Min/2, Max/2, Add3/2
  u_a/1 -> Add3/1
  Add1/1 -> Add6/1, Add5/1, Add4/1
  Add6/1 -> Relational Operator2/1
  Repeating Sequence/1 -> Relational Operator2/2, Relational Operator1/2, Relational Operator/2
  Constant7/1 -> Add6/2, Min/3, Max/3, Add2/2
  Add/1 -> Gain/1
  Add5/1 -> Relational Operator/1

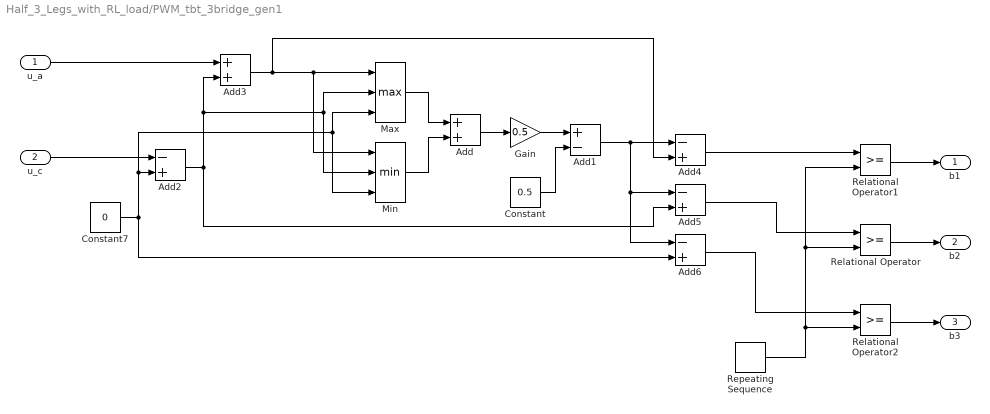
== system Half_3_Legs_with_RL_load/PWM_tbt_3bridge_gen1 ==
  u_a : Inport
  u_c : Inport  Port=2
  Add : Sum
  Add1 : Sum  Inputs=+-
  Add{2,4..6} (4 alike) : Sum  Inputs=-+
  Add3 : Sum
  Constant : Constant  Value=0.5
  Constant7 : Constant  Value=0
  Gain : Gain  Gain=0.5
  Max : MinMax  Function=max  Inputs=3
  Min : MinMax  Inputs=3
  Relational Operator : RelationalOperator  OutDataTypeStr=boolean  RndMeth=Simplest  InputSameDT=off
  Relational Operator1 : RelationalOperator  OutDataTypeStr=boolean  RndMeth=Simplest  InputSameDT=off
  Relational Operator2 : RelationalOperator  OutDataTypeStr=boolean  RndMeth=Simplest  InputSameDT=off
  Repeating Sequence : simulink/Sources/Repeating Sequence  rep_seq_t=[0 half_SW_Ts SW_Ts]  rep_seq_y=[0 1 0]
  b1 : Outport
  b2 : Outport  Port=2
  b3 : Outport  Port=3
  wires:
  Add4/1 -> Relational Operator1/1
  Max/1 -> Add/1
  Gain/1 -> Add1/1
  u_c/1 -> Add2/1
  Relational Operator2/1 -> b3/1
  Min/1 -> Add/2
  Relational Operator1/1 -> b1/1
  Constant/1 -> Add1/2
  Add3/1 -> Add4/2, Min/1, Max/1
  Relational Operator/1 -> b2/1
  Add2/1 -> Add5/2, Min/2, Max/2, Add3/2
  u_a/1 -> Add3/1
  Add1/1 -> Add6/1, Add5/1, Add4/1
  Add6/1 -> Relational Operator2/1
  Repeating Sequence/1 -> Relational Operator2/2, Relational Operator1/2, Relational Operator/2
  Constant7/1 -> Add6/2, Min/3, Max/3, Add2/2
  Add/1 -> Gain/1
  Add5/1 -> Relational Operator/1

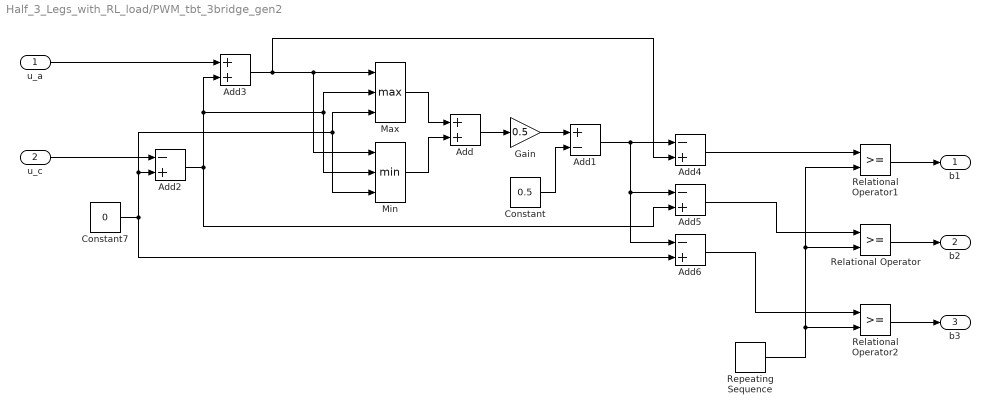
== system Half_3_Legs_with_RL_load/PWM_tbt_3bridge_gen2 ==
  u_a : Inport
  u_c : Inport  Port=2
  Add : Sum
  Add1 : Sum  Inputs=+-
  Add{2,4..6} (4 alike) : Sum  Inputs=-+
  Add3 : Sum
  Constant : Constant  Value=0.5
  Constant7 : Constant  Value=0
  Gain : Gain  Gain=0.5
  Max : MinMax  Function=max  Inputs=3
  Min : MinMax  Inputs=3
  Relational Operator : RelationalOperator  OutDataTypeStr=boolean  RndMeth=Simplest  InputSameDT=off
  Relational Operator1 : RelationalOperator  OutDataTypeStr=boolean  RndMeth=Simplest  InputSameDT=off
  Relational Operator2 : RelationalOperator  OutDataTypeStr=boolean  RndMeth=Simplest  InputSameDT=off
  Repeating Sequence : simulink/Sources/Repeating Sequence  rep_seq_t=[0 half_SW_Ts SW_Ts]  rep_seq_y=[0 1 0]
  b1 : Outport
  b2 : Outport  Port=2
  b3 : Outport  Port=3
  wires:
  Add4/1 -> Relational Operator1/1
  Max/1 -> Add/1
  Gain/1 -> Add1/1
  u_c/1 -> Add2/1
  Relational Operator2/1 -> b3/1
  Min/1 -> Add/2
  Relational Operator1/1 -> b1/1
  Constant/1 -> Add1/2
  Add3/1 -> Add4/2, Min/1, Max/1
  Relational Operator/1 -> b2/1
  Add2/1 -> Add5/2, Min/2, Max/2, Add3/2
  u_a/1 -> Add3/1
  Add1/1 -> Add6/1, Add5/1, Add4/1
  Add6/1 -> Relational Operator2/1
  Repeating Sequence/1 -> Relational Operator2/2, Relational Operator1/2, Relational Operator/2
  Constant7/1 -> Add6/2, Min/3, Max/3, Add2/2
  Add/1 -> Gain/1
  Add5/1 -> Relational Operator/1

== system Half_3_Legs_with_RL_load/SW_btb_3bridge_gen ==
  b1 : Inport
  b2 : Inport  Port=2
  b3 : Inport  Port=3
  Gain1 : Gain  Gain=15  OutDataTypeStr=double
  Gain2 : Gain  Gain=15  OutDataTypeStr=double
  Gain3 : Gain  Gain=15  OutDataTypeStr=double
  Logical Operator : Logic  Operator=NOT  AllPortsSameDT=off  OutDataTypeStr=boolean
  Logical Operator1 : Logic  Operator=NOT  AllPortsSameDT=off  OutDataTypeStr=boolean
  sw1 : Outport
  sw2 : Outport  Port=2
  sw3 : Outport  Port=3
  wires:
  b2/1 -> Gain2/1
  Gain1/1 -> sw3/1
  b3/1 -> Logical Operator1/1
  b1/1 -> Logical Operator/1
  Gain3/1 -> sw1/1
  Gain2/1 -> sw2/1
  Logical Operator/1 -> Gain3/1
  Logical Operator1/1 -> Gain1/1

== system Half_3_Legs_with_RL_load/SW_btb_3bridge_gen1 ==
  b1 : Inport
  b2 : Inport  Port=2
  b3 : Inport  Port=3
  Gain1 : Gain  Gain=15  OutDataTypeStr=double
  Gain2 : Gain  Gain=15  OutDataTypeStr=double
  Gain3 : Gain  Gain=15  OutDataTypeStr=double
  Logical Operator : Logic  Operator=NOT  AllPortsSameDT=off  OutDataTypeStr=boolean
  Logical Operator1 : Logic  Operator=NOT  AllPortsSameDT=off  OutDataTypeStr=boolean
  sw1 : Outport
  sw2 : Outport  Port=2
  sw3 : Outport  Port=3
  wires:
  b2/1 -> Gain2/1
  Gain1/1 -> sw3/1
  b3/1 -> Logical Operator1/1
  b1/1 -> Logical Operator/1
  Gain3/1 -> sw1/1
  Gain2/1 -> sw2/1
  Logical Operator/1 -> Gain3/1
  Logical Operator1/1 -> Gain1/1

== system Half_3_Legs_with_RL_load/SW_tbt_3bridge_gen ==
  b1 : Inport
  b2 : Inport  Port=2
  b3 : Inport  Port=3
  Gain1 : Gain  Gain=15  OutDataTypeStr=double
  Gain2 : Gain  Gain=15  OutDataTypeStr=double
  Gain3 : Gain  Gain=15  OutDataTypeStr=double
  Logical Operator : Logic  Operator=NOT  AllPortsSameDT=off  OutDataTypeStr=boolean
  sw1 : Outport
  sw2 : Outport  Port=2
  sw3 : Outport  Port=3
  wires:
  Logical Operator/1 -> Gain2/1
  b2/1 -> Logical Operator/1
  Gain1/1 -> sw3/1
  b3/1 -> Gain1/1
  b1/1 -> Gain3/1
  Gain3/1 -> sw1/1
  Gain2/1 -> sw2/1

== system Half_3_Legs_with_RL_load/SW_tbt_3bridge_gen1 ==
  b1 : Inport
  b2 : Inport  Port=2
  b3 : Inport  Port=3
  Gain1 : Gain  Gain=15  OutDataTypeStr=double
  Gain2 : Gain  Gain=15  OutDataTypeStr=double
  Gain3 : Gain  Gain=15  OutDataTypeStr=double
  Logical Operator : Logic  Operator=NOT  AllPortsSameDT=off  OutDataTypeStr=boolean
  sw1 : Outport
  sw2 : Outport  Port=2
  sw3 : Outport  Port=3
  wires:
  Logical Operator/1 -> Gain2/1
  b2/1 -> Logical Operator/1
  Gain1/1 -> sw3/1
  b3/1 -> Gain1/1
  b1/1 -> Gain3/1
  Gain3/1 -> sw1/1
  Gain2/1 -> sw2/1

== system Half_3_Legs_with_RL_load/SW_tbt_3bridge_gen2 ==
  b1 : Inport
  b2 : Inport  Port=2
  b3 : Inport  Port=3
  Gain1 : Gain  Gain=15  OutDataTypeStr=double
  Gain2 : Gain  Gain=15  OutDataTypeStr=double
  Gain3 : Gain  Gain=15  OutDataTypeStr=double
  Logical Operator : Logic  Operator=NOT  AllPortsSameDT=off  OutDataTypeStr=boolean
  sw1 : Outport
  sw2 : Outport  Port=2
  sw3 : Outport  Port=3
  wires:
  Logical Operator/1 -> Gain2/1
  b2/1 -> Logical Operator/1
  Gain1/1 -> sw3/1
  b3/1 -> Gain1/1
  b1/1 -> Gain3/1
  Gain3/1 -> sw1/1
  Gain2/1 -> sw2/1
